simulink model "autocodePlant"  (R2026a)
settings: Solver=ode4
settings Model: DataDictionary=autocodePlantParams.sldd  Creator=Christian  LastModifiedBy=Christian
settings HardwareCC: ProdLargestAtomicInteger=Long  ProdLargestAtomicFloat=Double  ProdHWDeviceType=ARM Compatible->ARM Cortex-M7 (MPS2)
settings RTWCC: SystemTargetFile=ert.tlc  GenCodeOnly=on  Toolchain=GNU Tools for STM32  Description=Embedded Coder
settings CodeAppCC: CustomSymbolStrMacro=$R_$N$M
settings ERTTargetCC: UtilityFuncGeneration=Shared location  GenerateSampleERTMain=on  CodeInterfacePackaging=Reusable function  SupportContinuousTime=on

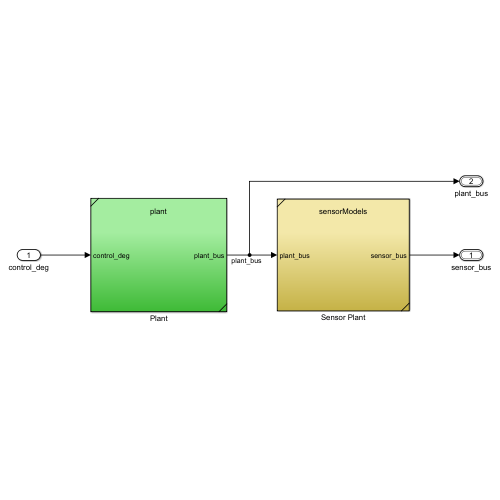
[thumbnail: Simulink's stored preview of the top-level diagram]
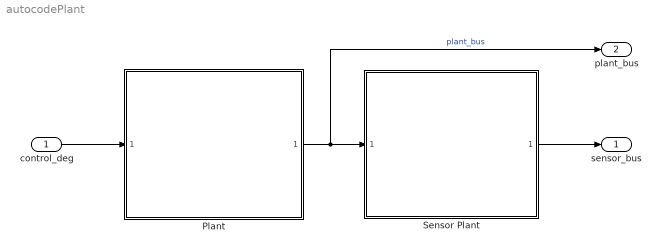
== system autocodePlant ==
  control_deg : Inport
  Plant : Subsystem  ReferencedSubsystem=plant
      settings: PermitHierarchicalResolution=None
  Sensor Plant : Subsystem  ReferencedSubsystem=sensorModels
      settings: PermitHierarchicalResolution=None
  sensor_bus : Outport  OutDataTypeStr=Bus: sensor_bus
  plant_bus : Outport  Port=2  OutDataTypeStr=Bus: plant_bus
  wires:
  Plant/1 -> plant_bus/1, Sensor Plant/1  "plant_bus"
  control_deg/1 -> Plant/1
  Sensor Plant/1 -> sensor_bus/1
